simulink model "cll_zcs_ver_v"  (R2026b)
settings: Solver=ode23tb  StopTime=simlength  FixedStep=tc  MaxStep=tc  EnableMultiTasking=on
PostLoadFcn:
  | if any(exist('dsrtsu_mdlpostloadfcn', 'file') ~= 0), dsrtsu_mdlpostloadfcn('Execute', bdroot); end
InitFcn:
  | , if any(exist('rtifpga_mdlclblib', 'file') ~= 0), rtifpga_mdlclblib('Init', bdroot); end,
  | , if any(exist('dsmpb_private', 'file') ~= 0), dsmpb_private('dsmpb_mdlclblib', 'Init', bdroot); end,
values from neighbouring files (symbols this model uses):
  Adrso = eye(2) + Arso*ts    [init_zcs_model_ctrl.m]
  Adrsoh = eye(2) + Arsoh*ts    [init_zcs_model_ctrl.m]
  Crso = [1 0]    [init_zcs_model_ctrl.m]
  Crsoh = [1 0]    [init_zcs_model_ctrl.m]
  fres = 1/2/pi/sqrt(Cs*(Ls+L1sigma))    [init_zcs_model_ctrl.m]
  I_FS = Iout_dc_nom * margin_factor    (= 125)    [init_zcs_model_ctrl.m]
  Iout_ref_SI = 100*scale    (= 100)    [init_zcs_model_ctrl.m]
  k_h10_comp = -12    [init_zcs_model_ctrl.m]
  k_h12_comp = -12    [init_zcs_model_ctrl.m]
  k_h14_comp = -12    [init_zcs_model_ctrl.m]
  k_h2_comp = -12    [init_zcs_model_ctrl.m]
  k_h4_comp = -12    [init_zcs_model_ctrl.m]
  k_h6_comp = -12    [init_zcs_model_ctrl.m]
  k_h8_comp = -12    [init_zcs_model_ctrl.m]
  ki_i_zcs = 80    [init_zcs_model_ctrl.m]
  ki_v_zcs = 80    [init_zcs_model_ctrl.m]
  kp_i_zcs = 0.25    [init_zcs_model_ctrl.m]
  kp_v_zcs = 0.25    [init_zcs_model_ctrl.m]
  Ldrso = acker(Adrso',Crso',polesdrso)'    [init_zcs_model_ctrl.m]
  Ldrsoh = acker(Adrsoh',Crsoh',polesdrsoh)'    [init_zcs_model_ctrl.m]
  omega_grid_emu_nom = w_grid    (= 314.159265359)    [grid_emulator.m]
  omega_grid_nom = w_grid    (= 314.159265359)    [grid_emulator.m]
  pll_i1 = 80    [init_zcs_model_ctrl.m]
  pll_p = 1    [init_zcs_model_ctrl.m]
  q1kalman = ts/10    (= 1e-05)    [init_zcs_model_ctrl.m]
  q2kalman = ts/10    (= 1e-05)    [init_zcs_model_ctrl.m]
  Rkalman = 1/ts    (= 10000)    [init_zcs_model_ctrl.m]
  tc = 1e-7    (= 1e-07)    [init_zcs_model_ctrl.m]
  ts = 1e-4    (= 0.0001)    [init_zcs_model_ctrl.m]
  V_FS = Vout_dc_nom * margin_factor    (= 12.5)    [init_zcs_model_ctrl.m]
  V_phase_normalization_factor = Vgrid_phase_normalization_factor    [grid_emulator.m]
  Vgrid_phase_normalization_factor = Vphase2*sqrt(2)    [grid_emulator.m]
  vn_eta_pu = 0.05    [init_zcs_model_ctrl.m]
  vn_xi_pu = 0.05    [init_zcs_model_ctrl.m]
  Vout_dc_nom = 10    [init_zcs_model_ctrl.m]
  vp_xi_pu = 0.9    [init_zcs_model_ctrl.m]
undefined symbols (not defined in the file or in its folder): magnitude
libraries: fl_lib x55, nesl_utility x18, cstblocks_lti x7, single_phase_transformer_lib x1
(part 1 of 2)
CloseFcn:
  | , if any(exist('dsmpb_private', 'file') ~= 0), dsmpb_private('dsmpb_mdlclblib', 'Close', bdroot); end,
PreSaveFcn:
  | , if any(exist('dsmpb_private', 'file') ~= 0), dsmpb_private('dsmpb_mdlclblib', 'PreSave', bdroot); end,
settings Model: DSRTSU_INTERNAL_RTIFPGA=170  DSRTSU_INTERNAL_RTISTBM_VER=1.4.3  RTICANMMDATA=struct('GeneralSetupData',struct('modelroot','C:\Users\dabagnara\Dropbox\anno_2022_2023\matlab\anno2022\alintel_cll_resonant\2022_08_31','generalsettings',struct('filesettings',struct('destfolder',struct('Name','RTICANMM_FILES','Check',1),'buildfolder',struct('Name','.','Check',1),'AbsDestfolder',struct('Name','C:\Users\dabagnara\Dropbox\anno_2022_2023\matlab\anno2022\alintel_cll_resonant\2022_08_31\RTICANMM_FILES'),'AbsBuildfolder',struct('Name','C:\Users\dabagnara\Dropbox\anno_2022_2023\matlab\anno2022\alintel_cll_resonant\2022_08_31'))),'options',struct('addpaths',1,'rmpaths',1,'addtrcexclusion',true,'cannavigator',struct('checkmonitoring',0),'show_usrtrc',0,'use_usrtrc',0),'advanced',struct('options',ones(1,100)),'MPSetup',{{}},'RTI',struct('Type','ERT','Ver','','Date',''),'modelname','cll_zcs_ver_i','block','cll_zcs_ver_i'))  Creator=LTNBDA  LastModifiedBy=d.bagnara
settings SolverCC: AutoInsertRateTranBlk=on  SolverResetMethod=Robust  ZeroCrossAlgorithm=Adaptive  ZeroCrossControl=EnableAll
settings DataIOCC: DSMLogging=off  LimitDataPoints=on  MaxDataPoints=1  ReturnWorkspaceOutputs=off  SaveFormat=Array  SaveOutput=off  SaveTime=off  SignalLogging=off  SignalLoggingSaveFormat=ModelDataLogs
settings OptimizationCC: BlockReduction=off  ConditionallyExecuteInputs=off  DefaultParameterBehavior=Inlined  DifferentSizesBufferReuse=on  EfficientMapNaN2IntZero=off  EfficientTunableParamExpr=on  EnhancedBackFolding=on  MemsetInitFltsAndDblsToZero=off  OptimizationCustomize=off  OptimizeBlockOrder=speed  PassReuseOutputArgsAs=Individual arguments  RemoveInternalMemoryZeroInit=on  RemoveRootLevelIOMemoryZeroInit=on
settings DebuggingCC: ArithmeticOperatorsInVariantConditions=warning  FcnCallInpInsideContextMsg=warning  MergeDetectMultiDrivingBlocksExec=none  MultiTaskCondExecSysMsg=none  MultiTaskDSMMsg=warning  ParameterTunabilityLossMsg=error  SFNoUnconditionalDefaultTransitionDiag=warning  SFUnexpectedBacktrackingDiag=warning  SaveWithParameterizedLinksMsg=none  SignalResolutionControl=TryResolveAllWithWarning  SolverPrmCheckMsg=warning  StateNameClashWarn=warning  TasksWithSamePriorityMsg=none  UnderspecifiedInitializationDetection=Classic
settings HardwareCC: ProdHWDeviceType=Custom Processor->Custom  ProdLargestAtomicInteger=Integer  ProdLongLongMode=on  TargetEndianess=LittleEndian  TargetHWDeviceType=MATLAB Host  TargetIntDivRoundTo=Zero  TargetLongLongMode=on
settings ModelReferenceCC: EnableParallelModelReferenceBuilds=on  PropagateSignalLabelsOutOfModel=off
settings SFSimCC: CustomCodeUndefinedFunction=UseInterfaceOnly  MATLABDynamicMemAlloc=off  SimDebugExecutionForCustomCode=on  SimParseCustomCode=off  SimUseLocalCustomCode=off
settings RTWCC: Description=Embedded Coder  GenCodeOnly=on  RTWUseLocalCustomCode=off  RTWVerbose=off  SystemTargetFile=ert.tlc  TemplateMakefile=ert_default_tmf
settings CodeAppCC: ForceParamTrailComments=on  IgnoreCustomStorageClasses=off  InsertBlockDesc=on  OperatorAnnotations=on  SFDataObjDesc=on  SimulinkDataObjDesc=on
settings ERTTargetCC: DynamicArrayContainerType=coder::array  GenerateSampleERTMain=on
settings ConfigComp: CovExternalEMLEnable=off  CovSaveCumulativeToWorkspaceVar=on  CovSaveSingleToWorkspaceVar=on
settings SimscapeCC: SimscapeNormalizeSystem=off  SimscapeUseEnergyAccounting=off

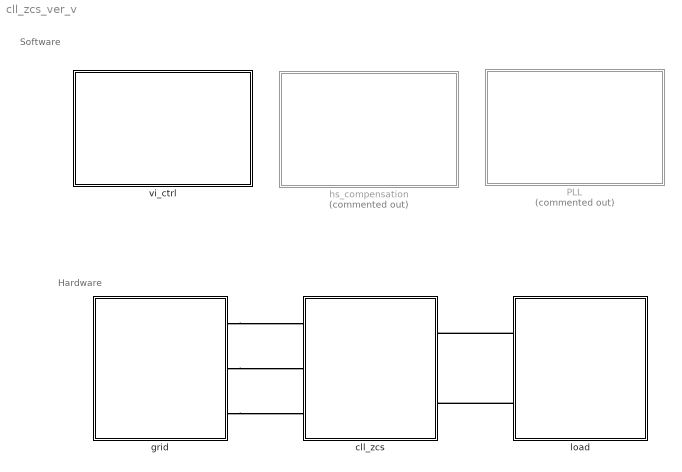
== system cll_zcs_ver_v ==
  note: Hardware
  note: Software
  PLL : Subsystem  Commented=on
  cll_zcs : Subsystem
  grid : Subsystem
  hs_compensation : Subsystem  Commented=on
  load : Subsystem
  vi_ctrl : Subsystem
  connections:
  grid/RConn1 -- cll_zcs/LConn1
  load/LConn1 -- cll_zcs/RConn1
  grid/RConn2 -- cll_zcs/LConn2
  load/LConn2 -- cll_zcs/RConn2
  grid/RConn3 -- cll_zcs/LConn3

== system cll_zcs_ver_v/PLL ==
  note: PLL
  pll_stageA : Subsystem
  pll_stageB : Subsystem
  tag scope: gamma_grid=global
  wires:
  pll_stageB/1(wt_grid) -> [gamma_grid], pll_stageA/1(gamma_grid)
  pll_stageA/2(u_grid_pos_eta) -> pll_stageB/2(u_grid_pos_eta)  "u_grid_pos_eta"
  pll_stageA/1(u_grid_pos_xi) -> pll_stageB/1(u_grid_pos_xi)  "u_grid_pos_xi"

== system cll_zcs_ver_v/cll_zcs ==
  HBridge : Subsystem
  LCtank : Subsystem
  grid_rectifier : Subsystem
  rectifier_RCfilter : Subsystem
  single phase transformer : single_phase_transformer_lib/single phase transformer  Lm=Lm_trafo H  n1=n1  n2=n2  Rd1=Rd1_trafo Ohm  Rd2=Rd2_trafo Ohm  Ld1=Ld1_trafo H  Ld2=Ld2_trafo H  Rfe=R0_trafo Ohm  phi_specify=off  phi_priority=None  phi=0 V*s  phi_nominal_specify=off  phi_nominal_value=1  phi_nominal_unit=V*s  i1_specify=off  i1_priority=None  i1=0 A  i1_nominal_specify=off  i1_nominal_value=1  i1_nominal_unit=A  i2_specify=off  i2_priority=None  i2=0 A  i2_nominal_specify=off  i2_nominal_value=1  i2_nominal_unit=A  ife_specify=off  ife_priority=None  ife=0 A  ife_nominal_specify=off  ife_nominal_value=1  ife_nominal_unit=A  u1_specify=off  u1_priority=None  u1=0 V  u1_nominal_specify=off  u1_nominal_value=1  u1_nominal_unit=V  u2_specify=off  u2_priority=None  u2=0 V  u2_nominal_specify=off  u2_nominal_value=1  u2_nominal_unit=V
  U1 : PMIOPort  Side=Left
  dc1 : PMIOPort  Port=2  Side=Right
  U2 : PMIOPort  Port=3  Side=Left
  dc2 : PMIOPort  Port=4  Side=Right
  U3 : PMIOPort  Port=5  Side=Left
  connections:
  single phase transformer/RConn2 -- rectifier_RCfilter/LConn2
  U3/RConn1 -- grid_rectifier/LConn3
  grid_rectifier/RConn1 -- HBridge/LConn1
  single phase transformer/LConn2 -- LCtank/RConn2
  grid_rectifier/RConn2 -- HBridge/LConn2
  HBridge/RConn2 -- LCtank/LConn2
  single phase transformer/LConn1 -- LCtank/RConn1
  dc1/RConn1 -- rectifier_RCfilter/RConn1
  rectifier_RCfilter/LConn1 -- single phase transformer/RConn1
  HBridge/RConn1 -- LCtank/LConn1
  dc2/RConn1 -- rectifier_RCfilter/RConn2
  U1/RConn1 -- grid_rectifier/LConn1
  U2/RConn1 -- grid_rectifier/LConn2

== system cll_zcs_ver_v/grid ==
  To Workspace8 : ToWorkspace  VariableName=grid_vi_ts  SampleTime=ts
      settings: MaxDataPoints=Ns  Save2DSignal=2-D array (concatenate along first dimension)
  grid_emulator : Subsystem
  threephase_vi_measures : Subsystem
  ua : PMIOPort  Side=Right
  ub : PMIOPort  Port=2  Side=Right
  uc : PMIOPort  Port=3  Side=Right
  wires:
  threephase_vi_measures/1(iv_data) -> To Workspace8/1
  connections:
  threephase_vi_measures/LConn3 -- grid_emulator/RConn3
  threephase_vi_measures/LConn1 -- grid_emulator/RConn1
  threephase_vi_measures/RConn2 -- ub/RConn1
  threephase_vi_measures/LConn2 -- grid_emulator/RConn2
  threephase_vi_measures/RConn1 -- ua/RConn1
  threephase_vi_measures/RConn3 -- uc/RConn1

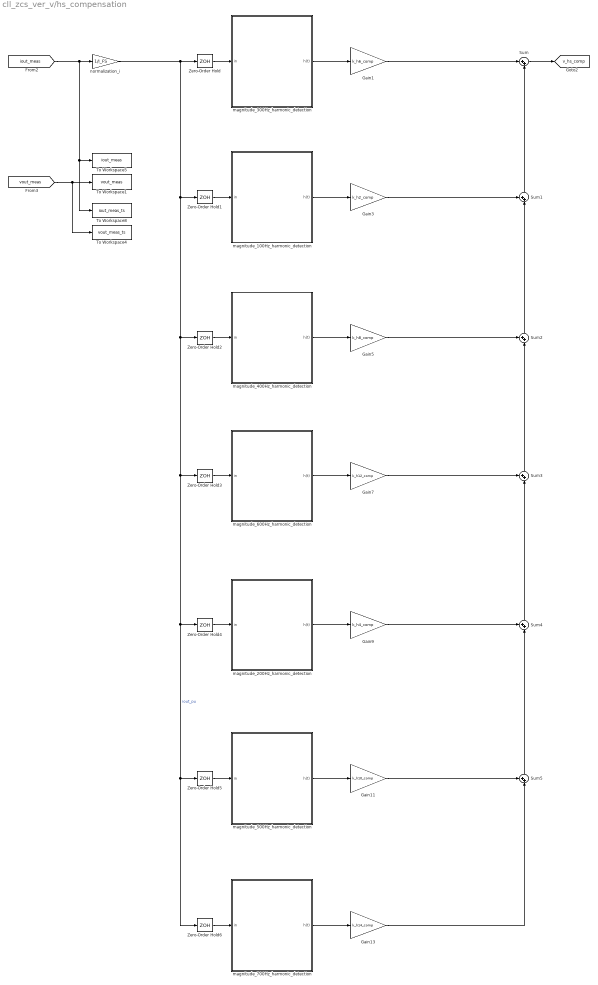
== system cll_zcs_ver_v/hs_compensation ==
  Gain1 : Gain  Gain=k_h6_comp
  Gain11 : Gain  Gain=k_h10_comp
  Gain13 : Gain  Gain=k_h14_comp
  Gain3 : Gain  Gain=k_h2_comp
  Gain5 : Gain  Gain=k_h8_comp
  Gain7 : Gain  Gain=k_h12_comp
  Gain9 : Gain  Gain=k_h4_comp
  Sum : Sum  Inputs=|++
  Sum{1..5} (5 alike) : Sum  Inputs=++|
  To Workspace1 : ToWorkspace  VariableName=vout_meas  SampleTime=tc
      settings: MaxDataPoints=Nc  Save2DSignal=2-D array (concatenate along first dimension)
  To Workspace4 : ToWorkspace  VariableName=vout_meas_ts  SampleTime=ts
      settings: MaxDataPoints=Ns  Save2DSignal=2-D array (concatenate along first dimension)
  To Workspace5 : ToWorkspace  VariableName=iout_meas  SampleTime=tc
      settings: MaxDataPoints=Nc  Save2DSignal=2-D array (concatenate along first dimension)
  To Workspace8 : ToWorkspace  VariableName=iout_meas_ts  SampleTime=ts
      settings: MaxDataPoints=Ns  Save2DSignal=2-D array (concatenate along first dimension)
  Zero-Order Hold{,1..6} (7 alike) : ZeroOrderHold  SampleTime=ts
  magnitude_100Hz_harmonic_detection : Subsystem
  magnitude_200Hz_harmonic_detection : Subsystem
  magnitude_300Hz_harmonic_detection : Subsystem
  magnitude_400Hz_harmonic_detection : Subsystem
  magnitude_500Hz_harmonic_detection : Subsystem
  magnitude_600Hz_harmonic_detection : Subsystem
  magnitude_700Hz_harmonic_detection : Subsystem
  normalization_i : Gain  Gain=1/I_FS  OutDataTypeStr=double  SaturateOnIntegerOverflow=on  ParamDataTypeStr=Inherit: Same as input
  tag scope: v_hs_comp=global
  wires:
  Zero-Order Hold1/1 -> magnitude_100Hz_harmonic_detection/1(in)
  Zero-Order Hold/1 -> magnitude_300Hz_harmonic_detection/1(in)
  [iout_meas] -> To Workspace8/1, To Workspace5/1, normalization_i/1
  [vout_meas] -> To Workspace4/1, To Workspace1/1
  Zero-Order Hold2/1 -> magnitude_400Hz_harmonic_detection/1(in)
  Sum1/1 -> Sum/2
  Zero-Order Hold3/1 -> magnitude_600Hz_harmonic_detection/1(in)
  Sum2/1 -> Sum1/2
  Zero-Order Hold4/1 -> magnitude_200Hz_harmonic_detection/1(in)
  Sum3/1 -> Sum2/2
  Sum/1 -> [v_hs_comp]
  Zero-Order Hold5/1 -> magnitude_500Hz_harmonic_detection/1(in)
  Sum4/1 -> Sum3/2
  normalization_i/1 -> Zero-Order Hold/1, Zero-Order Hold6/1, Zero-Order Hold5/1, Zero-Order Hold4/1, Zero-Order Hold3/1, Zero-Order Hold2/1, Zero-Order Hold1/1  "iout_pu"
  Zero-Order Hold6/1 -> magnitude_700Hz_harmonic_detection/1(in)
  Sum5/1 -> Sum4/2
  magnitude_600Hz_harmonic_detection/1(h(t)) -> Gain7/1
  Gain7/1 -> Sum3/1
  magnitude_400Hz_harmonic_detection/1(h(t)) -> Gain5/1
  Gain5/1 -> Sum2/1
  magnitude_100Hz_harmonic_detection/1(h(t)) -> Gain3/1
  Gain3/1 -> Sum1/1
  magnitude_300Hz_harmonic_detection/1(h(t)) -> Gain1/1
  Gain1/1 -> Sum/1
  magnitude_200Hz_harmonic_detection/1(h(t)) -> Gain9/1
  Gain9/1 -> Sum4/1
  magnitude_500Hz_harmonic_detection/1(h(t)) -> Gain11/1
  Gain11/1 -> Sum5/1
  magnitude_700Hz_harmonic_detection/1(h(t)) -> Gain13/1
  Gain13/1 -> Sum5/2

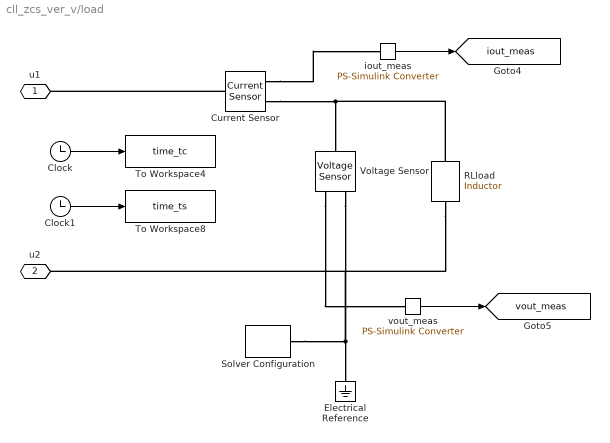
== system cll_zcs_ver_v/load ==
  Clock : Clock
  Clock1 : Clock
  Current Sensor : fl_lib/Electrical/Electrical Sensors/Current Sensor
  Electrical Reference : fl_lib/Electrical/Electrical Elements/Electrical Reference
  RLload : fl_lib/Electrical/Electrical Elements/Inductor  l=Lload H  r=Rload Ohm  g=1e-9 1/Ohm  i_specify=off  i_priority=None  i=0 A  i_nominal_specify=off  i_nominal_value=1  i_nominal_unit=A  v_specify=off  v_priority=None  v=0 V  v_nominal_specify=off  v_nominal_value=1  v_nominal_unit=V  i_L_specify=off  i_L_priority=High  i_L=0 A  i_L_nominal_specify=off  i_L_nominal_value=1  i_L_nominal_unit=A
  Solver Configuration : nesl_utility/Solver Configuration  PhysicalDomain=network_engine_domain  SubClassName=solver  LeftPortType=input  RightPortType=generic  Tones=[]  Harmonics=[]  SimulateNoise=off  Profile=off  UseLocalSampling=off  EnableSwitchedLinearOptims=on  FrequencyDomain=off  UseCCode=off  RelTol=0.001  AbsTol=0.001  MinStep=1e-09  ToWorkspace=off  RevertToSquareIcSolve=off  NumHomotopyIterations=100  PhasorMode=off  PhasorModeNumHarmonics=1  ConsistencySolver=NEWTON_FTOL  CanonicalOrdering=UNORDERED  OptimizeIntermediates=UNOPTIMIZED  MulticoreSolverChoice=BACKWARD_EULER  IndexReductionMethod=DerivativeReplacement  DoDC=off  ResidualTolerance=1e-09  ConsistencyTolSource=GLOBAL  ConsistencyAbsTol=0.001  ConsistencyRelTol=0.001  ConsistencyTolFactor=0.001  UseLocalSolver=on  LocalSolverChoice=NE_BACKWARD_EULER_ADVANCER  ResolveIndetEquations=on  FunctionEvalNumThread=1  LocalSolverSampleTime=tc  DoFixedCost=on  MaxNonlinIter=3  MaxModeIter=2  ComputeImpulses=off  ImpulseIterations=2  LinearAlgebra=auto  LinearAlgebraNumThread=0  EquationFormulation=NE_TIME_EF  DelaysMemoryBudget=1024  AutomaticFiltering=on  FilteringTimeConstant=0.001  PartitionStorageMethod=AS_NEEDED  PartitionMemoryBudget=1024  PartitionMethod=BALANCED  MultibodyUseLocalSolver=off  MultibodyLocalSolverChoice=ODE1  MultibodyLocalSolverSampleTime=0.001
  To Workspace4 : ToWorkspace  VariableName=time_tc  SampleTime=tc
      settings: MaxDataPoints=Nc  Save2DSignal=2-D array (concatenate along first dimension)
  To Workspace8 : ToWorkspace  VariableName=time_ts  SampleTime=ts
      settings: MaxDataPoints=Ns  Save2DSignal=2-D array (concatenate along first dimension)
  Voltage Sensor : fl_lib/Electrical/Electrical Sensors/Voltage Sensor
  iout_meas : nesl_utility/PS-Simulink Converter  PhysicalDomain=network_engine_domain  SubClassName=ps_output  LeftPortType=input  RightPortType=output  PseudoPeriodic=off  Frequencies=[]  VectorFormat=1-D array  Unit=A  AffineConversion=on
  vout_meas : nesl_utility/PS-Simulink Converter  PhysicalDomain=network_engine_domain  SubClassName=ps_output  LeftPortType=input  RightPortType=output  PseudoPeriodic=off  Frequencies=[]  VectorFormat=1-D array  Unit=V  AffineConversion=on
  u1 : PMIOPort  Side=Left
  u2 : PMIOPort  Port=2  Side=Left
  tag scope: iout_meas=global, vout_meas=global
  wires:
  iout_meas/1 -> [iout_meas]
  vout_meas/1 -> [vout_meas]
  Clock/1 -> To Workspace4/1
  Clock1/1 -> To Workspace8/1
  connections:
  Current Sensor/RConn2 -- RLload/LConn1 -- Voltage Sensor/LConn1
  RLload/RConn1 -- Voltage Sensor/RConn2 -- u2/RConn1 -- Solver Configuration/RConn1 -- Electrical Reference/LConn1
  Current Sensor/LConn1 -- u1/RConn1
  Current Sensor/RConn1 -- iout_meas/LConn1
  Voltage Sensor/RConn1 -- vout_meas/LConn1

== system cll_zcs_ver_v/vi_ctrl ==
  modulator : Subsystem
  references : Subsystem
  sampling_i_filter1 : Subsystem
  sampling_v_filter1 : Subsystem
  sampling_v_filter2 : Subsystem
  vi ctrl : Subsystem
  tag scope: g1=global, g2=global
  wires:
  [vout_meas] -> sampling_v_filter1/1(in)
  [iout_meas] -> sampling_i_filter1/1(in)
  vi ctrl/1(freq_ctrl_out) -> modulator/1(freq_ctrl_out)
  sampling_i_filter1/1(out_pu) -> vi ctrl/1(iout)
  sampling_v_filter1/1(out_pu) -> vi ctrl/2(vout)
  sampling_v_filter2/1(out_pu) -> vi ctrl/3(vout_ref)
  references/1(vout_ref) -> sampling_v_filter2/1(in)
  modulator/1(m_gA) -> [g1]
  modulator/2(m_gB) -> [g2]

== system cll_zcs_ver_v/PLL/pll_stageA ==
  gamma_grid : Inport
  Demux : Demux  Outputs=3
  Math Function : Math  Operator=magnitude^2  SignedPower=on
  Math Function1 : Math  Operator=magnitude^2  SignedPower=on
  Reciprocal Sqrt : Sqrt  Operator=rSqrt
  Saturation : Saturate  UpperLimit=inf  LowerLimit=0.02
  Sum : Sum  Inputs=|++
  mormalization_and_transformation : Subsystem
  sequences : Subsystem
  u_grid_pos_xi : Outport  VectorParamsAs1DForOutWhenUnconnected=off
  u_grid_pos_eta : Outport  Port=2  VectorParamsAs1DForOutWhenUnconnected=off
  tag scope: Vgrid_unorm=global
  wires:
  Saturation/1 -> Reciprocal Sqrt/1
  Reciprocal Sqrt/1 -> [Vgrid_unorm]
  Sum/1 -> Saturation/1
  Math Function1/1 -> Sum/2
  Math Function/1 -> Sum/1
  mormalization_and_transformation/2(ug_beta) -> sequences/2(u_grid_beta), Math Function1/1
  mormalization_and_transformation/1(ug_alpha) -> sequences/1(u_grid_alpha), Math Function/1
  Demux/3 -> mormalization_and_transformation/3(ug_c)
  Demux/2 -> mormalization_and_transformation/2(ug_b)
  Demux/1 -> mormalization_and_transformation/1(ug_a)
  [Vgrid] -> Demux/1
  sequences/1(u_grid_pos_xi) -> u_grid_pos_xi/1
  sequences/2(u_grid_pos_eta) -> u_grid_pos_eta/1
  gamma_grid/1 -> sequences/3(phase_angle)

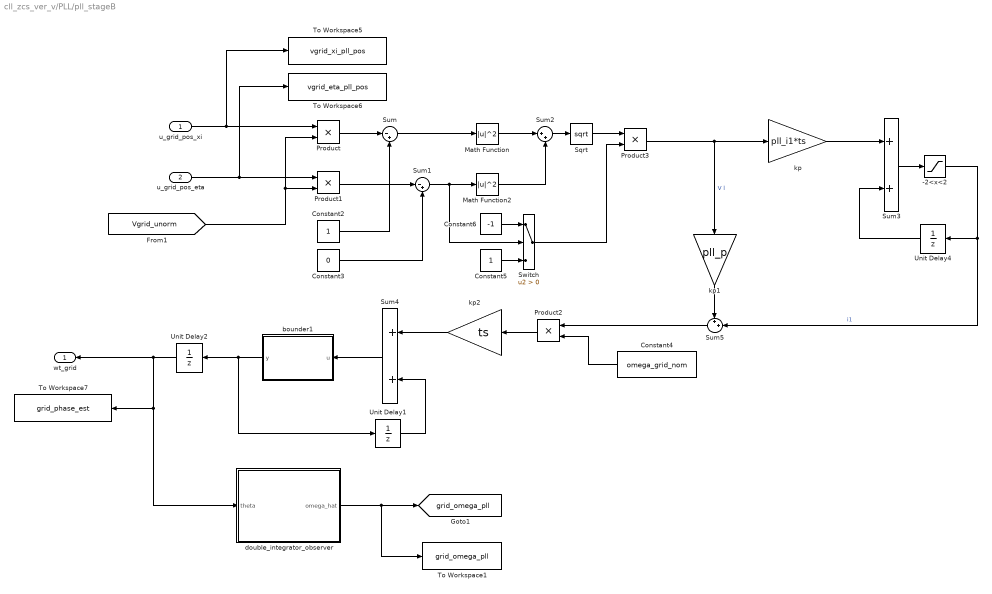
== system cll_zcs_ver_v/PLL/pll_stageB ==
  u_grid_pos_xi : Inport
  u_grid_pos_eta : Inport  Port=2
  -2<x<2 : Saturate  UpperLimit=2  LowerLimit=-2
  Constant2 : Constant
  Constant3 : Constant  Value=0
  Constant4 : Constant  Value=omega_grid_nom
  Constant5 : Constant
  Constant6 : Constant  Value=-1
  Math Function : Math  Operator=magnitude^2  SignedPower=on
  Math Function2 : Math  Operator=magnitude^2  SignedPower=on
  Product{,1..3} (4 alike) : Product  RndMeth=Zero
  Sqrt : Sqrt
  Sum : Sum  Inputs=|-+
  Sum1 : Sum  Inputs=|-+
  Sum2 : Sum  Inputs=|++
  Sum3 : Sum  SaturateOnIntegerOverflow=on
  Sum4 : Sum  SaturateOnIntegerOverflow=on
  Sum5 : Sum  Inputs=++|
  Switch : Switch  Criteria=u2 > Threshold  SampleTime=ts  SaturateOnIntegerOverflow=off  InputSameDT=off
  To Workspace1 : ToWorkspace  VariableName=grid_omega_pll  SampleTime=ts
      settings: MaxDataPoints=Ns
  To Workspace5 : ToWorkspace  VariableName=vgrid_xi_pll_pos  SampleTime=ts
      settings: MaxDataPoints=Ns
  To Workspace6 : ToWorkspace  VariableName=vgrid_eta_pll_pos  SampleTime=ts
      settings: MaxDataPoints=Ns
  To Workspace7 : ToWorkspace  VariableName=grid_phase_est  SampleTime=ts
      settings: MaxDataPoints=Ns
  Unit Delay1 : UnitDelay  SampleTime=ts
  Unit Delay2 : UnitDelay  SampleTime=ts
  Unit Delay4 : UnitDelay  SampleTime=ts
  bounder1 : MATLAB Function  TreatAsAtomicUnit=on  SystemSampleTime=ts
  double_integrator_observer : Subsystem
  kp : Gain  Gain=pll_i1*ts  SaturateOnIntegerOverflow=on  OutDataTypeStr=Inherit: Same as input  ParamDataTypeStr=Inherit: Same as input
  kp1 : Gain  Gain=pll_p  SaturateOnIntegerOverflow=on  OutDataTypeStr=Inherit: Same as input  ParamDataTypeStr=Inherit: Same as input
  kp2 : Gain  Gain=ts  SaturateOnIntegerOverflow=on  OutDataTypeStr=Inherit: Same as input  ParamDataTypeStr=Inherit: Same as input
  wt_grid : Outport  VectorParamsAs1DForOutWhenUnconnected=off
  tag scope: grid_omega_pll=global
  wires:
  Unit Delay2/1 -> wt_grid/1, double_integrator_observer/1(theta), To Workspace7/1
  kp1/1 -> Sum5/1
  Product3/1 -> kp1/1, kp/1  "V l"
  Product2/1 -> kp2/1
  u_grid_pos_eta/1 -> Product1/1, To Workspace6/1
  u_grid_pos_xi/1 -> To Workspace5/1, Product/1
  bounder1/1(y) -> Unit Delay1/1, Unit Delay2/1
  Sum5/1 -> Product2/1
  kp/1 -> Sum3/1
  Switch/1 -> Product3/2
  Sqrt/1 -> Product3/1
  Constant6/1 -> Switch/1
  Constant5/1 -> Switch/3
  [Vgrid_unorm] -> Product1/2, Product/2
  Constant4/1 -> Product2/2
  kp2/1 -> Sum4/1
  -2<x<2/1 -> Unit Delay4/1, Sum5/2  "i1"
  Unit Delay1/1 -> Sum4/2
  Sum4/1 -> bounder1/1(u)
  Sum3/1 -> -2<x<2/1
  Unit Delay4/1 -> Sum3/2
  Sum1/1 -> Math Function2/1, Switch/2
  Sum/1 -> Math Function/1
  Sum2/1 -> Sqrt/1
  Math Function2/1 -> Sum2/2
  Math Function/1 -> Sum2/1
  Constant3/1 -> Sum1/2
  Product1/1 -> Sum1/1
  Constant2/1 -> Sum/2
  Product/1 -> Sum/1
  double_integrator_observer/1(omega_hat) -> To Workspace1/1, [grid_omega_pll]

== system cll_zcs_ver_v/cll_zcs/HBridge ==
  C1 : fl_lib/Electrical/Electrical Elements/Capacitor  c=C1 F  r=RC1 Ohm  g=0 1/Ohm  i_specify=off  i_priority=None  i=0 A  i_nominal_specify=off  i_nominal_value=1  i_nominal_unit=A  v_specify=off  v_priority=None  v=0 V  v_nominal_specify=off  v_nominal_value=1  v_nominal_unit=V  vc_specify=off  vc_priority=High  vc=0 V  vc_nominal_specify=off  vc_nominal_value=1  vc_nominal_unit=V
  C2 : fl_lib/Electrical/Electrical Elements/Capacitor  c=C2 F  r=RC2 Ohm  g=0 1/Ohm  i_specify=off  i_priority=None  i=0 A  i_nominal_specify=off  i_nominal_value=1  i_nominal_unit=A  v_specify=off  v_priority=None  v=0 V  v_nominal_specify=off  v_nominal_value=1  v_nominal_unit=V  vc_specify=off  vc_priority=High  vc=0 V  vc_nominal_specify=off  vc_nominal_value=1  vc_nominal_unit=V
  switch_1 : Subsystem
      settings: PortSchema="{\"entries\":[{\"content\":{\"sides\":[{\"content\":{\"connectorIds\":[\"In1\"]},\"type\":\"ConnectorPlacement.EquallySpacedRectSide\",\"uuid\":\"4d0d9629-ddaf-4dec-8259-2fbb7f7a67ac\"},{\"content\":{\"connectorIds\":[],\"side\":\"RIGHT\"},\"type\":\"ConnectorPlacement.EquallySpacedRectSide\",\"uuid\":\"5762b4ea-aa37-4bba-a562-d5bb02789682\"},{\"content\":{\"connectorIds\":[\"LConn1\"],\"side\":\"TOP\"},\"type\":\"ConnectorPlacement.EquallySpacedRectSide\",\"uuid\":\"9177b3c9-154f-4d28-b5b3-70d5502d764f\"},{\"content\":{\"connectorIds\":[\"RConn1\"],\"side\":\"BOTTOM\"},\"type\":\"ConnectorPlacement.EquallySpacedRectSide\",\"uuid\":\"4020e1dd-2a2b-4451-9d71-800cc6f349cc\"}]},\"type\":\"ConnectorPlacement.EquallySpacedConnector\",\"uuid\":\"1666cebf-2867-4186-b78b-78922f63d994\"}],\"packageUris\":[\"http://schema.mathworks.com/mf0/Connector/R2020b\"],\"version\":\"1.0\"}"
  switch_2 : Subsystem
      settings: PortSchema="{\"entries\":[{\"content\":{\"sides\":[{\"content\":{\"connectorIds\":[\"In1\"]},\"type\":\"ConnectorPlacement.EquallySpacedRectSide\",\"uuid\":\"4d0d9629-ddaf-4dec-8259-2fbb7f7a67ac\"},{\"content\":{\"connectorIds\":[],\"side\":\"RIGHT\"},\"type\":\"ConnectorPlacement.EquallySpacedRectSide\",\"uuid\":\"5762b4ea-aa37-4bba-a562-d5bb02789682\"},{\"content\":{\"connectorIds\":[\"LConn1\"],\"side\":\"TOP\"},\"type\":\"ConnectorPlacement.EquallySpacedRectSide\",\"uuid\":\"9177b3c9-154f-4d28-b5b3-70d5502d764f\"},{\"content\":{\"connectorIds\":[\"RConn1\"],\"side\":\"BOTTOM\"},\"type\":\"ConnectorPlacement.EquallySpacedRectSide\",\"uuid\":\"4020e1dd-2a2b-4451-9d71-800cc6f349cc\"}]},\"type\":\"ConnectorPlacement.EquallySpacedConnector\",\"uuid\":\"1666cebf-2867-4186-b78b-78922f63d994\"}],\"packageUris\":[\"http://schema.mathworks.com/mf0/Connector/R2020b\"],\"version\":\"1.0\"}"
  dc1 : PMIOPort  Side=Left
  dc2 : PMIOPort  Port=2  Side=Left
  u1 : PMIOPort  Port=3  Side=Right
  u2 : PMIOPort  Port=4  Side=Right
  wires:
  [g2] -> switch_2/1(g)
  [g1] -> switch_1/1(g)
  connections:
  switch_1/LConn1 -- C1/LConn1 -- dc1/RConn1
  switch_2/LConn1 -- u1/RConn1 -- switch_1/RConn1
  switch_2/RConn1 -- C2/RConn1 -- dc2/RConn1
  u2/RConn1 -- C2/LConn1 -- C1/RConn1

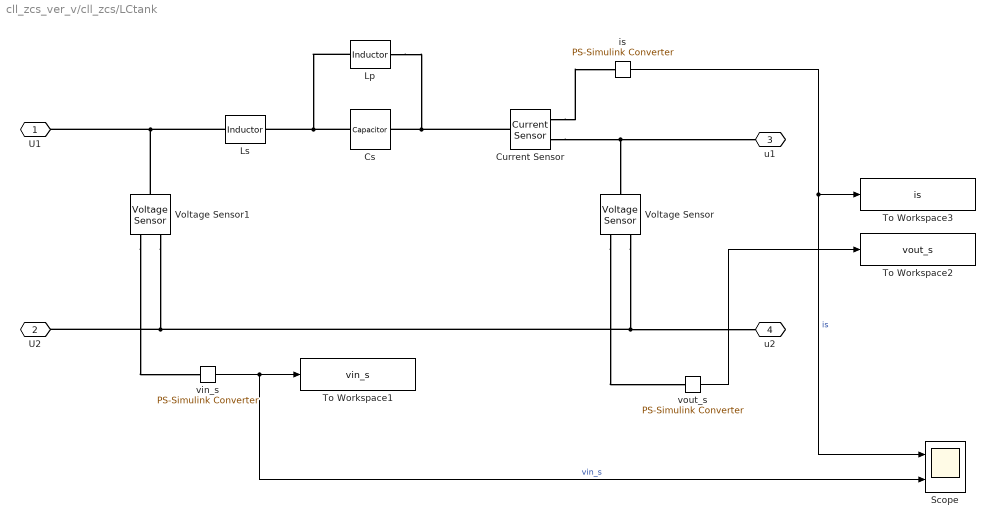
== system cll_zcs_ver_v/cll_zcs/LCtank ==
  Cs : fl_lib/Electrical/Electrical Elements/Capacitor  c=Cs F  r=RCs Ohm  g=0 1/Ohm  i_specify=off  i_priority=None  i=0 A  i_nominal_specify=off  i_nominal_value=1  i_nominal_unit=A  v_specify=off  v_priority=None  v=0 V  v_nominal_specify=off  v_nominal_value=1  v_nominal_unit=V  vc_specify=off  vc_priority=High  vc=0 V  vc_nominal_specify=off  vc_nominal_value=1  vc_nominal_unit=V
  Current Sensor : fl_lib/Electrical/Electrical Sensors/Current Sensor
  Lp : fl_lib/Electrical/Electrical Elements/Inductor  l=Lp H  r=RLp Ohm  g=0 1/Ohm  i_specify=off  i_priority=None  i=0 A  i_nominal_specify=off  i_nominal_value=1  i_nominal_unit=A  v_specify=off  v_priority=None  v=0 V  v_nominal_specify=off  v_nominal_value=1  v_nominal_unit=V  i_L_specify=off  i_L_priority=High  i_L=0 A  i_L_nominal_specify=off  i_L_nominal_value=1  i_L_nominal_unit=A
  Ls : fl_lib/Electrical/Electrical Elements/Inductor  l=Ls H  r=RLs Ohm  g=0 1/Ohm  i_specify=off  i_priority=None  i=0 A  i_nominal_specify=off  i_nominal_value=1  i_nominal_unit=A  v_specify=off  v_priority=None  v=0 V  v_nominal_specify=off  v_nominal_value=1  v_nominal_unit=V  i_L_specify=off  i_L_priority=High  i_L=0 A  i_L_nominal_specify=off  i_L_nominal_value=1  i_L_nominal_unit=A
  Scope : Scope  NumInputPorts=2
      settings: ActiveDisplayYMinimum=-347.8764880222451  ActiveDisplayYMaximum=347.21109478202686
  To Workspace1 : ToWorkspace  VariableName=vin_s  SampleTime=tc
      settings: MaxDataPoints=Nc  Save2DSignal=2-D array (concatenate along first dimension)
  To Workspace2 : ToWorkspace  VariableName=vout_s  SampleTime=tc
      settings: MaxDataPoints=Nc  Save2DSignal=2-D array (concatenate along first dimension)
  To Workspace3 : ToWorkspace  VariableName=is  SampleTime=tc
      settings: MaxDataPoints=Nc  Save2DSignal=2-D array (concatenate along first dimension)
  Voltage Sensor : fl_lib/Electrical/Electrical Sensors/Voltage Sensor
  Voltage Sensor1 : fl_lib/Electrical/Electrical Sensors/Voltage Sensor
  is : nesl_utility/PS-Simulink Converter  PhysicalDomain=network_engine_domain  SubClassName=ps_output  LeftPortType=input  RightPortType=output  PseudoPeriodic=off  Frequencies=[]  VectorFormat=1-D array  Unit=A  AffineConversion=on
  vin_s : nesl_utility/PS-Simulink Converter  PhysicalDomain=network_engine_domain  SubClassName=ps_output  LeftPortType=input  RightPortType=output  PseudoPeriodic=off  Frequencies=[]  VectorFormat=1-D array  Unit=V  AffineConversion=on
  vout_s : nesl_utility/PS-Simulink Converter  PhysicalDomain=network_engine_domain  SubClassName=ps_output  LeftPortType=input  RightPortType=output  PseudoPeriodic=off  Frequencies=[]  VectorFormat=1-D array  Unit=V  AffineConversion=on
  U1 : PMIOPort  Side=Left
  U2 : PMIOPort  Port=2  Side=Left
  u1 : PMIOPort  Port=3  Side=Right
  u2 : PMIOPort  Port=4  Side=Right
  wires:
  is/1 -> Scope/1, To Workspace3/1  "is"
  vout_s/1 -> To Workspace2/1
  vin_s/1 -> Scope/2, To Workspace1/1  "vin_s"
  connections:
  Lp/RConn1 -- Current Sensor/LConn1 -- Cs/RConn1
  Ls/LConn1 -- Voltage Sensor1/LConn1 -- U1/RConn1
  Cs/LConn1 -- Lp/LConn1 -- Ls/RConn1
  Voltage Sensor/RConn2 -- Voltage Sensor1/RConn2 -- U2/RConn1 -- u2/RConn1
  Current Sensor/RConn2 -- Voltage Sensor/LConn1 -- u1/RConn1
  Voltage Sensor/RConn1 -- vout_s/LConn1
  Current Sensor/RConn1 -- is/LConn1
  Voltage Sensor1/RConn1 -- vin_s/LConn1

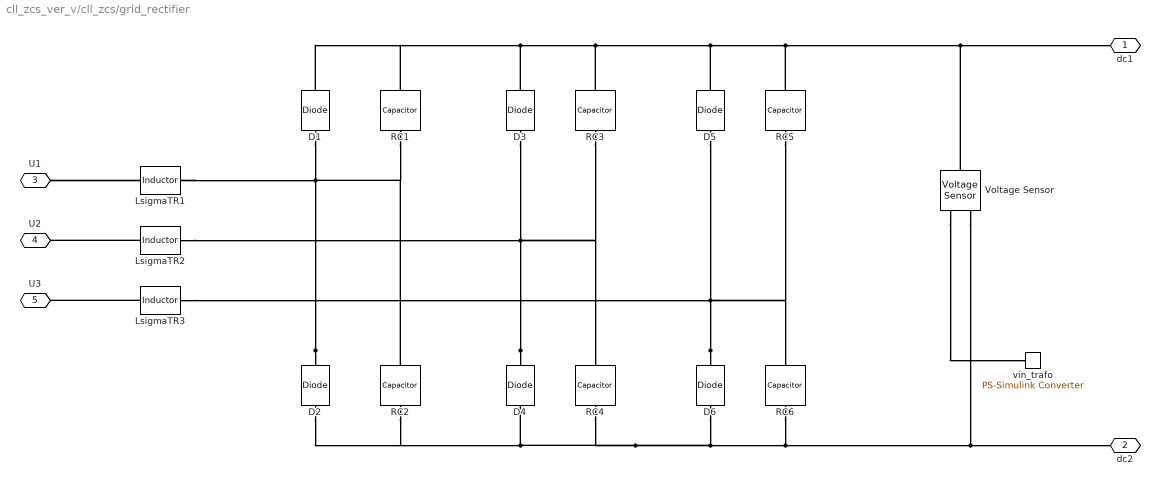
== system cll_zcs_ver_v/cll_zcs/grid_rectifier ==
  D{1..6} (6 alike) : fl_lib/Electrical/Electrical Elements/Diode  Vf=0.6 V  Ron=1e-3 Ohm  Goff=1e-8 1/Ohm  i_specify=off  i_priority=None  i=0 A  i_nominal_specify=off  i_nominal_value=1  i_nominal_unit=A  v_specify=off  v_priority=None  v=0 V  v_nominal_specify=off  v_nominal_value=1  v_nominal_unit=V
  LsigmaTR1 : fl_lib/Electrical/Electrical Elements/Inductor  l=LsigmaTR1 H  r=Rd_TR1 Ohm  g=1e-9 1/Ohm  i_specify=off  i_priority=None  i=0 A  i_nominal_specify=off  i_nominal_value=1  i_nominal_unit=A  v_specify=off  v_priority=None  v=0 V  v_nominal_specify=off  v_nominal_value=1  v_nominal_unit=V  i_L_specify=off  i_L_priority=High  i_L=0 A  i_L_nominal_specify=off  i_L_nominal_value=1  i_L_nominal_unit=A
  LsigmaTR2 : fl_lib/Electrical/Electrical Elements/Inductor  l=LsigmaTR1 H  r=Rd_TR1 Ohm  g=1e-9 1/Ohm  i_specify=off  i_priority=None  i=0 A  i_nominal_specify=off  i_nominal_value=1  i_nominal_unit=A  v_specify=off  v_priority=None  v=0 V  v_nominal_specify=off  v_nominal_value=1  v_nominal_unit=V  i_L_specify=off  i_L_priority=High  i_L=0 A  i_L_nominal_specify=off  i_L_nominal_value=1  i_L_nominal_unit=A
  LsigmaTR3 : fl_lib/Electrical/Electrical Elements/Inductor  l=LsigmaTR1 H  r=Rd_TR1 Ohm  g=1e-9 1/Ohm  i_specify=off  i_priority=None  i=0 A  i_nominal_specify=off  i_nominal_value=1  i_nominal_unit=A  v_specify=off  v_priority=None  v=0 V  v_nominal_specify=off  v_nominal_value=1  v_nominal_unit=V  i_L_specify=off  i_L_priority=High  i_L=0 A  i_L_nominal_specify=off  i_L_nominal_value=1  i_L_nominal_unit=A
  RC{1..6} (6 alike) : fl_lib/Electrical/Electrical Elements/Capacitor  c=Csnubber F  r=Rsnubber Ohm  g=0 1/Ohm  i_specify=off  i_priority=None  i=0 A  i_nominal_specify=off  i_nominal_value=1  i_nominal_unit=A  v_specify=off  v_priority=None  v=0 V  v_nominal_specify=off  v_nominal_value=1  v_nominal_unit=V  vc_specify=off  vc_priority=High  vc=0 V  vc_nominal_specify=off  vc_nominal_value=1  vc_nominal_unit=V
  Voltage Sensor : fl_lib/Electrical/Electrical Sensors/Voltage Sensor
  vin_trafo : nesl_utility/PS-Simulink Converter  PhysicalDomain=network_engine_domain  SubClassName=ps_output  LeftPortType=input  RightPortType=output  PseudoPeriodic=off  Frequencies=[]  VectorFormat=1-D array  Unit=V  AffineConversion=on
  dc1 : PMIOPort  Side=Right
  dc2 : PMIOPort  Port=2  Side=Right
  U1 : PMIOPort  Port=3  Side=Left
  U2 : PMIOPort  Port=4  Side=Left
  U3 : PMIOPort  Port=5  Side=Left
  connections:
  RC3/LConn1 -- D3/RConn1 -- RC1/LConn1 -- D1/RConn1 -- D5/RConn1 -- RC5/LConn1 -- Voltage Sensor/LConn1 -- dc1/RConn1
  RC4/RConn1 -- D4/LConn1 -- D2/LConn1 -- RC2/RConn1 -- D6/LConn1 -- RC6/RConn1 -- Voltage Sensor/RConn2 -- dc2/RConn1
  D4/RConn1 -- LsigmaTR2/RConn1 -- RC3/RConn1 -- RC4/LConn1 -- D3/LConn1
  D2/RConn1 -- LsigmaTR1/RConn1 -- RC1/RConn1 -- RC2/LConn1 -- D1/LConn1
  D6/RConn1 -- LsigmaTR3/RConn1 -- D5/LConn1 -- RC5/RConn1 -- RC6/LConn1
  Voltage Sensor/RConn1 -- vin_trafo/LConn1
  U1/RConn1 -- LsigmaTR1/LConn1
  LsigmaTR2/LConn1 -- U2/RConn1
  LsigmaTR3/LConn1 -- U3/RConn1

== system cll_zcs_ver_v/cll_zcs/rectifier_RCfilter ==
  Bleeder : fl_lib/Electrical/Electrical Elements/Resistor  R=1.5 Ohm  i_specify=off  i_priority=None  i=0 A  i_nominal_specify=off  i_nominal_value=1  i_nominal_unit=A  v_specify=off  v_priority=None  v=0 V  v_nominal_specify=off  v_nominal_value=1  v_nominal_unit=V
  CFu : fl_lib/Electrical/Electrical Elements/Capacitor  c=CFu F  r=RCFu Ohm  g=0 1/Ohm  i_specify=off  i_priority=None  i=0 A  i_nominal_specify=off  i_nominal_value=1  i_nominal_unit=A  v_specify=off  v_priority=None  v=0 V  v_nominal_specify=off  v_nominal_value=1  v_nominal_unit=V  vc_specify=off  vc_priority=High  vc=0 V  vc_nominal_specify=off  vc_nominal_value=1  vc_nominal_unit=V
  D{1..4} (4 alike) : fl_lib/Electrical/Electrical Elements/Diode  Vf=0.6 V  Ron=1e-3 Ohm  Goff=1e-8 1/Ohm  i_specify=off  i_priority=None  i=0 A  i_nominal_specify=off  i_nominal_value=1  i_nominal_unit=A  v_specify=off  v_priority=None  v=0 V  v_nominal_specify=off  v_nominal_value=1  v_nominal_unit=V
  RC{1..4} (4 alike) : fl_lib/Electrical/Electrical Elements/Capacitor  c=Csnubber F  r=Rsnubber Ohm  g=0 1/Ohm  i_specify=off  i_priority=None  i=0 A  i_nominal_specify=off  i_nominal_value=1  i_nominal_unit=A  v_specify=off  v_priority=None  v=0 V  v_nominal_specify=off  v_nominal_value=1  v_nominal_unit=V  vc_specify=off  vc_priority=High  vc=0 V  vc_nominal_specify=off  vc_nominal_value=1  vc_nominal_unit=V
  dc1 : PMIOPort  Side=Right
  dc2 : PMIOPort  Port=2  Side=Right
  u1 : PMIOPort  Port=3  Side=Left
  u2 : PMIOPort  Port=4  Side=Left
  connections:
  D1/LConn1 -- u1/RConn1 -- RC2/LConn1 -- RC1/RConn1 -- D2/RConn1
  D3/LConn1 -- u2/RConn1 -- RC3/RConn1 -- RC4/LConn1 -- D4/RConn1
  RC2/RConn1 -- D2/LConn1 -- RC4/RConn1 -- Bleeder/RConn1 -- CFu/RConn1 -- dc2/RConn1 -- D4/LConn1
  D1/RConn1 -- RC1/LConn1 -- D3/RConn1 -- RC3/LConn1 -- Bleeder/LConn1 -- CFu/LConn1 -- dc1/RConn1

== system cll_zcs_ver_v/grid/grid_emulator ==
  Controlled Voltage Source : fl_lib/Electrical/Electrical Sources/Controlled Voltage Source
  Controlled Voltage Source1 : fl_lib/Electrical/Electrical Sources/Controlled Voltage Source
  Controlled Voltage Source2 : fl_lib/Electrical/Electrical Sources/Controlled Voltage Source
  Electrical Reference : fl_lib/Electrical/Electrical Elements/Electrical Reference
  Simulink-PS Converter : nesl_utility/Simulink-PS Converter  PhysicalDomain=network_engine_domain  SubClassName=ps_input  LeftPortType=input  RightPortType=output  PseudoPeriodic=off  Frequencies=[]  NoiseDistribution=none  NoiseParameters=[]  Unit=V  AffineConversion=on  FilteringAndDerivatives=provide  SimscapeFilterOrder=1  InputFilterTimeConstant=0.001  UdotUserProvided=0
  Simulink-PS Converter1 : nesl_utility/Simulink-PS Converter  PhysicalDomain=network_engine_domain  SubClassName=ps_input  LeftPortType=input  RightPortType=output  PseudoPeriodic=off  Frequencies=[]  NoiseDistribution=none  NoiseParameters=[]  Unit=V  AffineConversion=on  FilteringAndDerivatives=provide  SimscapeFilterOrder=1  InputFilterTimeConstant=0.001  UdotUserProvided=0
  Simulink-PS Converter2 : nesl_utility/Simulink-PS Converter  PhysicalDomain=network_engine_domain  SubClassName=ps_input  LeftPortType=input  RightPortType=output  PseudoPeriodic=off  Frequencies=[]  NoiseDistribution=none  NoiseParameters=[]  Unit=V  AffineConversion=on  FilteringAndDerivatives=provide  SimscapeFilterOrder=1  InputFilterTimeConstant=0.001  UdotUserProvided=0
  grid_emulator : Subsystem
  u1 : PMIOPort  Side=Right
  u2 : PMIOPort  Port=2  Side=Right
  u3 : PMIOPort  Port=3  Side=Right
  wires:
  grid_emulator/2(Vmb) -> Simulink-PS Converter1/1
  grid_emulator/3(Vmc) -> Simulink-PS Converter2/1
  grid_emulator/1(Vma) -> Simulink-PS Converter/1
  connections:
  Controlled Voltage Source/LConn1 -- u1/RConn1
  u2/RConn1 -- Controlled Voltage Source1/LConn1
  u3/RConn1 -- Controlled Voltage Source2/LConn1
  Simulink-PS Converter/RConn1 -- Controlled Voltage Source/RConn1
  Simulink-PS Converter1/RConn1 -- Controlled Voltage Source1/RConn1
  Simulink-PS Converter2/RConn1 -- Controlled Voltage Source2/RConn1
  Electrical Reference/LConn1 -- Controlled Voltage Source/RConn2 -- Controlled Voltage Source1/RConn2 -- Controlled Voltage Source2/RConn2

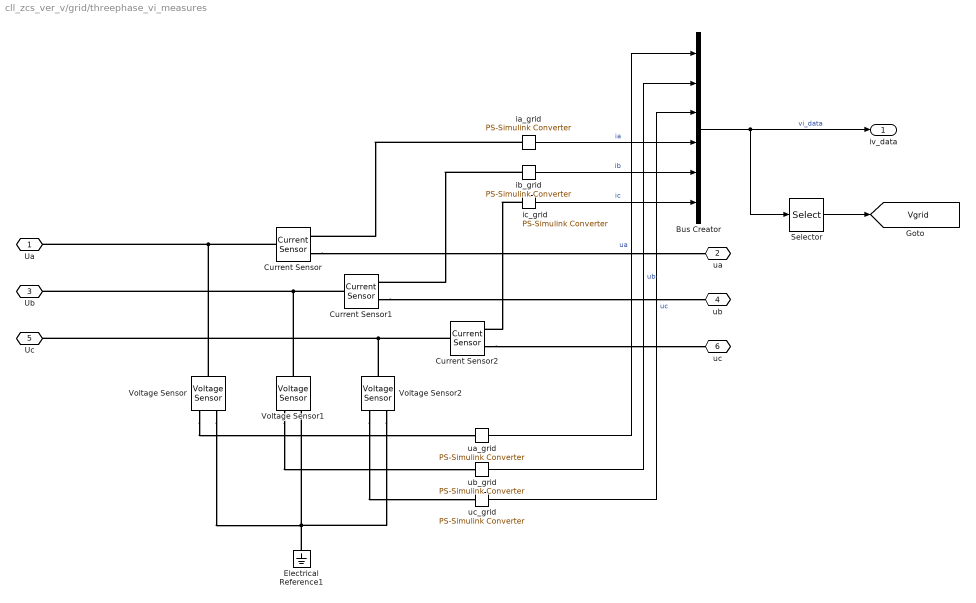
== system cll_zcs_ver_v/grid/threephase_vi_measures ==
  Bus Creator : BusCreator  Inputs=6
  Current Sensor : fl_lib/Electrical/Electrical Sensors/Current Sensor
  Current Sensor1 : fl_lib/Electrical/Electrical Sensors/Current Sensor
  Current Sensor2 : fl_lib/Electrical/Electrical Sensors/Current Sensor
  Electrical Reference1 : fl_lib/Electrical/Electrical Elements/Electrical Reference
  Selector : Selector  InputPortWidth=6  IndexOptions=Index vector (dialog)  Indices=[1 2 3]  OutputSizes=1  RuntimeRangeChecks=off
  Voltage Sensor : fl_lib/Electrical/Electrical Sensors/Voltage Sensor
  Voltage Sensor1 : fl_lib/Electrical/Electrical Sensors/Voltage Sensor
  Voltage Sensor2 : fl_lib/Electrical/Electrical Sensors/Voltage Sensor
  ia_grid : nesl_utility/PS-Simulink Converter  PhysicalDomain=network_engine_domain  SubClassName=ps_output  LeftPortType=input  RightPortType=output  PseudoPeriodic=off  Frequencies=[]  VectorFormat=1-D array  Unit=A  AffineConversion=on
  ib_grid : nesl_utility/PS-Simulink Converter  PhysicalDomain=network_engine_domain  SubClassName=ps_output  LeftPortType=input  RightPortType=output  PseudoPeriodic=off  Frequencies=[]  VectorFormat=1-D array  Unit=A  AffineConversion=on
  ic_grid : nesl_utility/PS-Simulink Converter  PhysicalDomain=network_engine_domain  SubClassName=ps_output  LeftPortType=input  RightPortType=output  PseudoPeriodic=off  Frequencies=[]  VectorFormat=1-D array  Unit=A  AffineConversion=on
  ua_grid : nesl_utility/PS-Simulink Converter  PhysicalDomain=network_engine_domain  SubClassName=ps_output  LeftPortType=input  RightPortType=output  PseudoPeriodic=off  Frequencies=[]  VectorFormat=1-D array  Unit=V  AffineConversion=on
  ub_grid : nesl_utility/PS-Simulink Converter  PhysicalDomain=network_engine_domain  SubClassName=ps_output  LeftPortType=input  RightPortType=output  PseudoPeriodic=off  Frequencies=[]  VectorFormat=1-D array  Unit=V  AffineConversion=on
  uc_grid : nesl_utility/PS-Simulink Converter  PhysicalDomain=network_engine_domain  SubClassName=ps_output  LeftPortType=input  RightPortType=output  PseudoPeriodic=off  Frequencies=[]  VectorFormat=1-D array  Unit=V  AffineConversion=on
  Ua : PMIOPort  Side=Left
  ua : PMIOPort  Port=2  Side=Right
  Ub : PMIOPort  Port=3  Side=Left
  ub : PMIOPort  Port=4  Side=Right
  Uc : PMIOPort  Port=5  Side=Left
  uc : PMIOPort  Port=6  Side=Right
  iv_data : Outport
  tag scope: Vgrid=global
  wires:
  Bus Creator/1 -> iv_data/1, Selector/1  "vi_data"
  Selector/1 -> [Vgrid]
  ib_grid/1 -> Bus Creator/5  "ib"
  ia_grid/1 -> Bus Creator/4  "ia"
  ic_grid/1 -> Bus Creator/6  "ic"
  ua_grid/1 -> Bus Creator/1  "ua"
  ub_grid/1 -> Bus Creator/2  "ub"
  uc_grid/1 -> Bus Creator/3  "uc"
  connections:
  Current Sensor1/LConn1 -- Ub/RConn1 -- Voltage Sensor1/LConn1
  Electrical Reference1/LConn1 -- Voltage Sensor/RConn2 -- Voltage Sensor2/RConn2 -- Voltage Sensor1/RConn2
  Voltage Sensor/RConn1 -- ua_grid/LConn1
  Current Sensor/RConn2 -- ua/RConn1
  Voltage Sensor1/RConn1 -- ub_grid/LConn1
  Voltage Sensor2/LConn1 -- Uc/RConn1 -- Current Sensor2/LConn1
  Current Sensor/LConn1 -- Ua/RConn1 -- Voltage Sensor/LConn1
  Current Sensor1/RConn2 -- ub/RConn1
  Voltage Sensor2/RConn1 -- uc_grid/LConn1
  ib_grid/LConn1 -- Current Sensor1/RConn1
  ia_grid/LConn1 -- Current Sensor/RConn1
  ic_grid/LConn1 -- Current Sensor2/RConn1
  Current Sensor2/RConn2 -- uc/RConn1

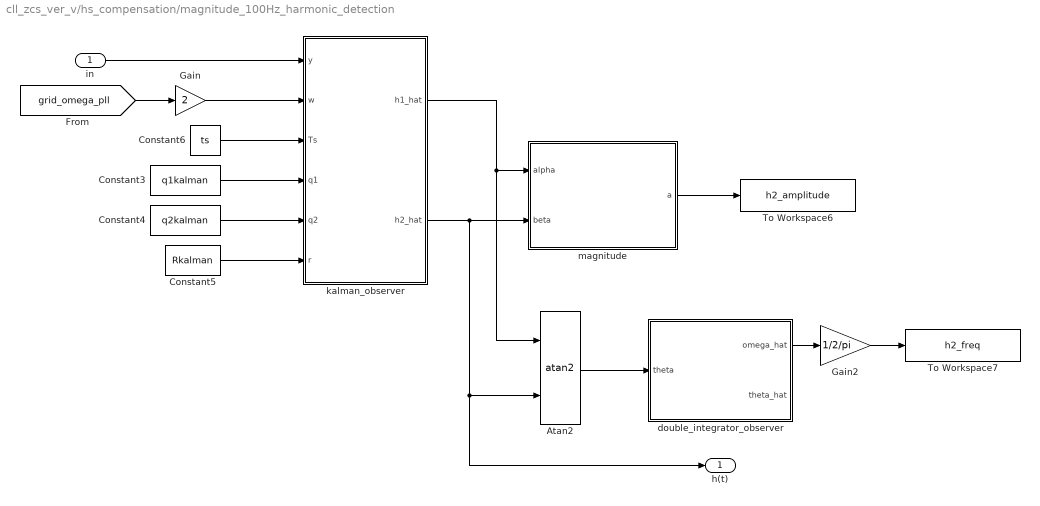
== system cll_zcs_ver_v/hs_compensation/magnitude_100Hz_harmonic_detection ==
  in : Inport
  Atan2 : Trigonometry  Operator=atan2
  Constant3 : Constant  Value=q1kalman
  Constant4 : Constant  Value=q2kalman
  Constant5 : Constant  Value=Rkalman
  Constant6 : Constant  Value=ts
  Gain : Gain  Gain=2
  Gain2 : Gain  Gain=1/2/pi
  To Workspace6 : ToWorkspace  VariableName=h2_amplitude  SampleTime=ts
      settings: MaxDataPoints=Ns  Save2DSignal=2-D array (concatenate along first dimension)
  To Workspace7 : ToWorkspace  VariableName=h2_freq  SampleTime=ts
      settings: MaxDataPoints=Ns  Save2DSignal=2-D array (concatenate along first dimension)
  double_integrator_observer : Subsystem
  kalman_observer : MATLAB Function  TreatAsAtomicUnit=on  SystemSampleTime=ts
  magnitude : Subsystem
  h(t) : Outport
  wires:
  Atan2/1 -> double_integrator_observer/1(theta)
  kalman_observer/1(h1_hat) -> Atan2/1, magnitude/1(alpha)
  Constant4/1 -> kalman_observer/5(q2)
  Constant3/1 -> kalman_observer/4(q1)
  Constant5/1 -> kalman_observer/6(r)
  Constant6/1 -> kalman_observer/3(Ts)
  in/1 -> kalman_observer/1(y)
  [grid_omega_pll] -> Gain/1
  Gain/1 -> kalman_observer/2(w)
  kalman_observer/2(h2_hat) -> h(t)/1, Atan2/2, magnitude/2(beta)
  double_integrator_observer/1(omega_hat) -> Gain2/1
  Gain2/1 -> To Workspace7/1
  magnitude/1(a) -> To Workspace6/1

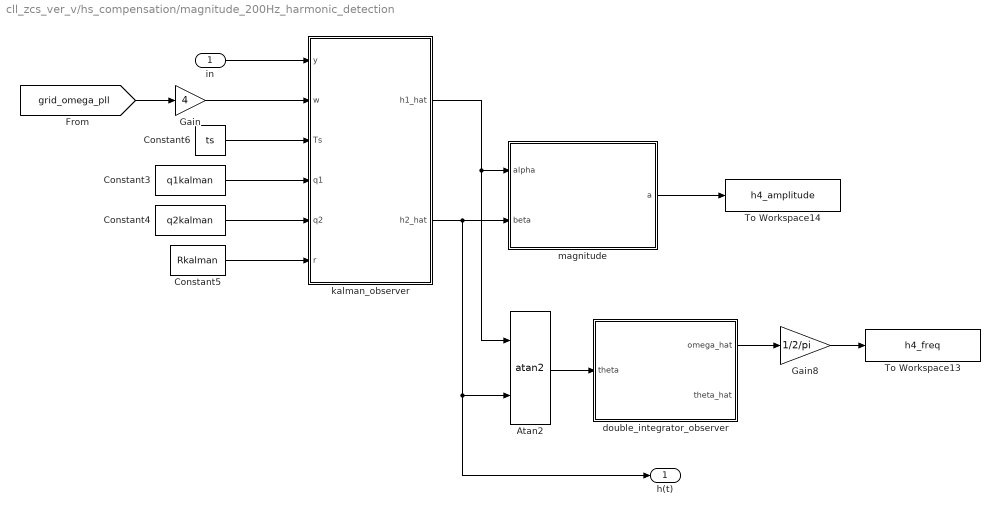
== system cll_zcs_ver_v/hs_compensation/magnitude_200Hz_harmonic_detection ==
  in : Inport
  Atan2 : Trigonometry  Operator=atan2
  Constant3 : Constant  Value=q1kalman
  Constant4 : Constant  Value=q2kalman
  Constant5 : Constant  Value=Rkalman
  Constant6 : Constant  Value=ts
  Gain : Gain  Gain=4
  Gain8 : Gain  Gain=1/2/pi
  To Workspace13 : ToWorkspace  VariableName=h4_freq  SampleTime=ts
      settings: MaxDataPoints=Ns  Save2DSignal=2-D array (concatenate along first dimension)
  To Workspace14 : ToWorkspace  VariableName=h4_amplitude  SampleTime=ts
      settings: MaxDataPoints=Ns  Save2DSignal=2-D array (concatenate along first dimension)
  double_integrator_observer : Subsystem
  kalman_observer : MATLAB Function  TreatAsAtomicUnit=on  SystemSampleTime=ts
  magnitude : Subsystem
  h(t) : Outport
  wires:
  in/1 -> kalman_observer/1(y)
  Constant6/1 -> kalman_observer/3(Ts)
  Constant5/1 -> kalman_observer/6(r)
  Constant3/1 -> kalman_observer/4(q1)
  Constant4/1 -> kalman_observer/5(q2)
  kalman_observer/1(h1_hat) -> Atan2/1, magnitude/1(alpha)
  Atan2/1 -> double_integrator_observer/1(theta)
  [grid_omega_pll] -> Gain/1
  Gain/1 -> kalman_observer/2(w)
  kalman_observer/2(h2_hat) -> h(t)/1, Atan2/2, magnitude/2(beta)
  double_integrator_observer/1(omega_hat) -> Gain8/1
  Gain8/1 -> To Workspace13/1
  magnitude/1(a) -> To Workspace14/1

== system cll_zcs_ver_v/hs_compensation/magnitude_300Hz_harmonic_detection ==
  in : Inport
  Atan2 : Trigonometry  Operator=atan2
  Constant3 : Constant  Value=q1kalman
  Constant4 : Constant  Value=q2kalman
  Constant5 : Constant  Value=Rkalman
  Constant6 : Constant  Value=ts
  Gain : Gain  Gain=6
  Gain1 : Gain  Gain=1/2/pi
  To Workspace2 : ToWorkspace  VariableName=h6_amplitude  SampleTime=ts
      settings: MaxDataPoints=Ns  Save2DSignal=2-D array (concatenate along first dimension)
  To Workspace3 : ToWorkspace  VariableName=h6_freq  SampleTime=ts
      settings: MaxDataPoints=Ns  Save2DSignal=2-D array (concatenate along first dimension)
  double_integrator_observer : Subsystem
  kalman_observer : MATLAB Function  TreatAsAtomicUnit=on  SystemSampleTime=ts
  magnitude : Subsystem
  h(t) : Outport
  wires:
  [grid_omega_pll] -> Gain/1
  in/1 -> kalman_observer/1(y)
  Constant6/1 -> kalman_observer/3(Ts)
  Constant5/1 -> kalman_observer/6(r)
  Constant3/1 -> kalman_observer/4(q1)
  Constant4/1 -> kalman_observer/5(q2)
  kalman_observer/1(h1_hat) -> Atan2/1, magnitude/1(alpha)
  kalman_observer/2(h2_hat) -> Atan2/2, h(t)/1, magnitude/2(beta)
  Atan2/1 -> double_integrator_observer/1(theta)
  Gain/1 -> kalman_observer/2(w)
  double_integrator_observer/1(omega_hat) -> Gain1/1
  magnitude/1(a) -> To Workspace2/1
  Gain1/1 -> To Workspace3/1

== system cll_zcs_ver_v/hs_compensation/magnitude_400Hz_harmonic_detection ==
  in : Inport
  Atan2 : Trigonometry  Operator=atan2
  Constant3 : Constant  Value=q1kalman
  Constant4 : Constant  Value=q2kalman
  Constant5 : Constant  Value=Rkalman
  Constant6 : Constant  Value=ts
  Gain : Gain  Gain=8
  Gain4 : Gain  Gain=1/2/pi
  To Workspace10 : ToWorkspace  VariableName=h8_freq  SampleTime=ts
      settings: MaxDataPoints=Ns  Save2DSignal=2-D array (concatenate along first dimension)
  To Workspace9 : ToWorkspace  VariableName=h8_amplitude  SampleTime=ts
      settings: MaxDataPoints=Ns  Save2DSignal=2-D array (concatenate along first dimension)
  double_integrator_observer : Subsystem
  kalman_observer : MATLAB Function  TreatAsAtomicUnit=on  SystemSampleTime=ts
  magnitude : Subsystem
  h(t) : Outport
  wires:
  in/1 -> kalman_observer/1(y)
  Constant6/1 -> kalman_observer/3(Ts)
  Constant5/1 -> kalman_observer/6(r)
  Constant3/1 -> kalman_observer/4(q1)
  Constant4/1 -> kalman_observer/5(q2)
  kalman_observer/1(h1_hat) -> Atan2/1, magnitude/1(alpha)
  Atan2/1 -> double_integrator_observer/1(theta)
  [grid_omega_pll] -> Gain/1
  Gain/1 -> kalman_observer/2(w)
  kalman_observer/2(h2_hat) -> h(t)/1, Atan2/2, magnitude/2(beta)
  double_integrator_observer/1(omega_hat) -> Gain4/1
  Gain4/1 -> To Workspace10/1
  magnitude/1(a) -> To Workspace9/1

== system cll_zcs_ver_v/hs_compensation/magnitude_500Hz_harmonic_detection ==
  in : Inport
  Atan2 : Trigonometry  Operator=atan2
  Constant3 : Constant  Value=q1kalman
  Constant4 : Constant  Value=q2kalman
  Constant5 : Constant  Value=Rkalman
  Constant6 : Constant  Value=ts
  Gain : Gain  Gain=10
  Gain10 : Gain  Gain=1/2/pi
  To Workspace15 : ToWorkspace  VariableName=h10_freq  SampleTime=ts
      settings: MaxDataPoints=Ns  Save2DSignal=2-D array (concatenate along first dimension)
  To Workspace16 : ToWorkspace  VariableName=h10_amplitude  SampleTime=ts
      settings: MaxDataPoints=Ns  Save2DSignal=2-D array (concatenate along first dimension)
  double_integrator_observer : Subsystem
  kalman_observer : MATLAB Function  TreatAsAtomicUnit=on  SystemSampleTime=ts
  magnitude : Subsystem
  h(t) : Outport
  wires:
  Atan2/1 -> double_integrator_observer/1(theta)
  kalman_observer/1(h1_hat) -> Atan2/1, magnitude/1(alpha)
  Constant4/1 -> kalman_observer/5(q2)
  Constant3/1 -> kalman_observer/4(q1)
  Constant5/1 -> kalman_observer/6(r)
  Constant6/1 -> kalman_observer/3(Ts)
  in/1 -> kalman_observer/1(y)
  [grid_omega_pll] -> Gain/1
  Gain/1 -> kalman_observer/2(w)
  kalman_observer/2(h2_hat) -> h(t)/1, Atan2/2, magnitude/2(beta)
  double_integrator_observer/1(omega_hat) -> Gain10/1
  Gain10/1 -> To Workspace15/1
  magnitude/1(a) -> To Workspace16/1

== system cll_zcs_ver_v/hs_compensation/magnitude_600Hz_harmonic_detection ==
  in : Inport
  Atan2 : Trigonometry  Operator=atan2
  Constant3 : Constant  Value=q1kalman
  Constant4 : Constant  Value=q2kalman
  Constant5 : Constant  Value=Rkalman
  Constant6 : Constant  Value=ts
  Gain : Gain  Gain=12
  Gain6 : Gain  Gain=1/2/pi
  To Workspace11 : ToWorkspace  VariableName=h12_freq  SampleTime=ts
      settings: MaxDataPoints=Ns  Save2DSignal=2-D array (concatenate along first dimension)
  To Workspace12 : ToWorkspace  VariableName=h12_amplitude  SampleTime=ts
      settings: MaxDataPoints=Ns  Save2DSignal=2-D array (concatenate along first dimension)
  double_integrator_observer : Subsystem
  kalman_observer : MATLAB Function  TreatAsAtomicUnit=on  SystemSampleTime=ts
  magnitude : Subsystem
  h(t) : Outport
  wires:
  Atan2/1 -> double_integrator_observer/1(theta)
  kalman_observer/1(h1_hat) -> Atan2/1, magnitude/1(alpha)
  Constant4/1 -> kalman_observer/5(q2)
  Constant3/1 -> kalman_observer/4(q1)
  Constant5/1 -> kalman_observer/6(r)
  Constant6/1 -> kalman_observer/3(Ts)
  in/1 -> kalman_observer/1(y)
  Gain/1 -> kalman_observer/2(w)
  [grid_omega_pll] -> Gain/1
  kalman_observer/2(h2_hat) -> h(t)/1, Atan2/2, magnitude/2(beta)
  double_integrator_observer/1(omega_hat) -> Gain6/1
  Gain6/1 -> To Workspace11/1
  magnitude/1(a) -> To Workspace12/1

== system cll_zcs_ver_v/hs_compensation/magnitude_700Hz_harmonic_detection ==
  in : Inport
  Atan2 : Trigonometry  Operator=atan2
  Constant3 : Constant  Value=q1kalman
  Constant4 : Constant  Value=q2kalman
  Constant5 : Constant  Value=Rkalman
  Constant6 : Constant  Value=ts
  Gain : Gain  Gain=14
  Gain12 : Gain  Gain=1/2/pi
  To Workspace17 : ToWorkspace  VariableName=h14_freq  SampleTime=ts
      settings: MaxDataPoints=Ns  Save2DSignal=2-D array (concatenate along first dimension)
  To Workspace18 : ToWorkspace  VariableName=h14_amplitude  SampleTime=ts
      settings: MaxDataPoints=Ns  Save2DSignal=2-D array (concatenate along first dimension)
  double_integrator_observer : Subsystem
  kalman_observer : MATLAB Function  TreatAsAtomicUnit=on  SystemSampleTime=ts
  magnitude : Subsystem
  h(t) : Outport
  wires:
  in/1 -> kalman_observer/1(y)
  Constant6/1 -> kalman_observer/3(Ts)
  Constant5/1 -> kalman_observer/6(r)
  Constant3/1 -> kalman_observer/4(q1)
  Constant4/1 -> kalman_observer/5(q2)
  kalman_observer/1(h1_hat) -> Atan2/1, magnitude/1(alpha)
  Atan2/1 -> double_integrator_observer/1(theta)
  [grid_omega_pll] -> Gain/1
  Gain/1 -> kalman_observer/2(w)
  kalman_observer/2(h2_hat) -> h(t)/1, Atan2/2, magnitude/2(beta)
  Gain12/1 -> To Workspace17/1
  double_integrator_observer/1(omega_hat) -> Gain12/1
  magnitude/1(a) -> To Workspace18/1

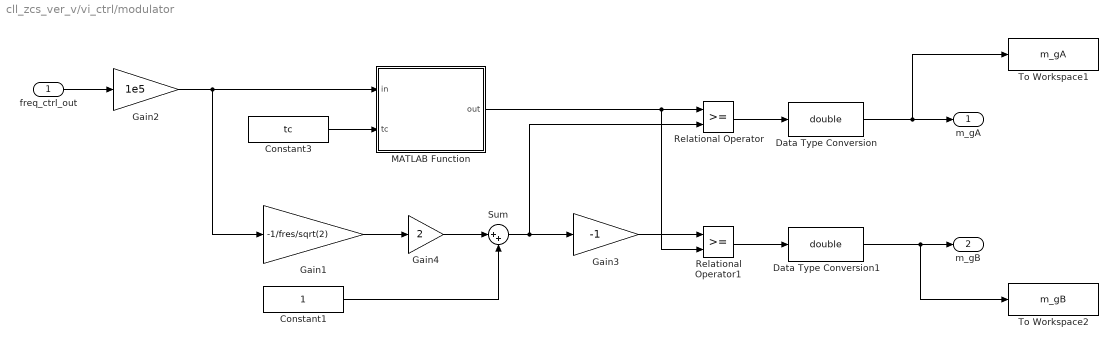
== system cll_zcs_ver_v/vi_ctrl/modulator ==
  freq_ctrl_out : Inport
  Constant1 : Constant
  Constant3 : Constant  Value=tc
  Data Type Conversion : DataTypeConversion  OutDataTypeStr=double  SaturateOnIntegerOverflow=off  RndMeth=Floor
  Data Type Conversion1 : DataTypeConversion  OutDataTypeStr=double  SaturateOnIntegerOverflow=off  RndMeth=Floor
  Gain1 : Gain  Gain=-1/fres/sqrt(2)  OutDataTypeStr=double
  Gain2 : Gain  Gain=1e5  OutDataTypeStr=double
  Gain3 : Gain  Gain=-1  OutDataTypeStr=double
  Gain4 : Gain  Gain=2  OutDataTypeStr=double
  MATLAB Function : MATLAB Function  TreatAsAtomicUnit=on  SystemSampleTime=tc
  Relational Operator : RelationalOperator
  Relational Operator1 : RelationalOperator
  Sum : Sum  Inputs=|++
  To Workspace1 : ToWorkspace  VariableName=m_gA  SampleTime=tc
      settings: MaxDataPoints=Nc  Save2DSignal=2-D array (concatenate along first dimension)
  To Workspace2 : ToWorkspace  VariableName=m_gB  SampleTime=tc
      settings: MaxDataPoints=Nc  Save2DSignal=2-D array (concatenate along first dimension)
  m_gA : Outport
  m_gB : Outport  Port=2
  wires:
  freq_ctrl_out/1 -> Gain2/1
  MATLAB Function/1(out) -> Relational Operator1/2, Relational Operator/1
  Constant3/1 -> MATLAB Function/2(tc)
  Relational Operator/1 -> Data Type Conversion/1
  Data Type Conversion/1 -> To Workspace1/1, m_gA/1
  Data Type Conversion1/1 -> To Workspace2/1, m_gB/1
  Gain2/1 -> Gain1/1, MATLAB Function/1(in)
  Gain1/1 -> Gain4/1
  Sum/1 -> Gain3/1, Relational Operator/2
  Constant1/1 -> Sum/2
  Gain3/1 -> Relational Operator1/1
  Relational Operator1/1 -> Data Type Conversion1/1
  Gain4/1 -> Sum/1

== system cll_zcs_ver_v/vi_ctrl/references ==
  voltage_reference : Subsystem
  vout_ref : Outport
  wires:
  voltage_reference/1(vout_ref) -> vout_ref/1

== system cll_zcs_ver_v/vi_ctrl/sampling_i_filter1 ==
  in : Inport
  1/Ti3 : Gain  Gain=1/I_FS  OutDataTypeStr=double  SaturateOnIntegerOverflow=on  ParamDataTypeStr=Inherit: Same as input
  Saturation : Saturate  UpperLimit=1  LowerLimit=0  OutDataTypeStr=double
  Zero-Order Hold2 : ZeroOrderHold  SampleTime=ts
  out_pu : Outport
  wires:
  in/1 -> 1/Ti3/1
  1/Ti3/1 -> Saturation/1
  Saturation/1 -> Zero-Order Hold2/1
  Zero-Order Hold2/1 -> out_pu/1
